simulink model "TWLan"  (R2025a)
settings: Solver=ode4  StartTime=0.0  StopTime=inf  FixedStep=0.01  RelTol=1e-3
libraries: AFCToolbox x9, simulink x3, etargetslib x2
settings Model: Creator=zqinghua  LastModifiedBy=zqhkd
settings OptimizationCC: DefaultParameterBehavior=Inlined  EnhancedBackFolding=on  PassReuseOutputArgsAs=Individual arguments  ZeroExternalMemoryAtStartup=off  ZeroInternalMemoryAtStartup=off  OptimizeBlockOrder=speed  DifferentSizesBufferReuse=on  OptimizationCustomize=off  EfficientTunableParamExpr=on
settings DebuggingCC: ParameterTunabilityLossMsg=error
settings HardwareCC: ProdBitPerInt=16.0  ProdBitPerPointer=16.0  ProdBitPerSizeT=16.0  ProdBitPerPtrDiffT=16.0  ProdLargestAtomicFloat=None  ProdWordSize=16.0  ProdHWDeviceType=STMicroelectronics->ST10/Super10
settings SFSimCC: MATLABDynamicMemAlloc=off
settings RTWCC: SystemTargetFile=AFCHawk.tlc  GenCodeOnly=on  TemplateMakefile=ert_default_tmf  GPUComputeCapability=3.5  Description=Embedded Coder
settings CodeAppCC: ForceParamTrailComments=on  IgnoreCustomStorageClasses=off  OperatorAnnotations=on  SimulinkDataObjDesc=on  SFDataObjDesc=on  InsertBlockDesc=on
settings STFCustomTargetCC: SystemTargetFile=AFCHawk.tlc  TargetLangStandard=C99 (ISO)  MultiwordLength=256.0  DynamicStringBufferSize=256.0  ModelReferenceCompliant=off  CombineOutputUpdateFcns=on  ERTCustomFileBanners=on  SupportContinuousTime=off  SupportNonInlinedSFcns=off  RemoveResetFunc=on  MATLABClassNameForMDSCustomization=Simulink.SoftwareTarget.ERTCustomization  GRTInterface=off  t_comPort=6.0  t_productKey=45638.0  t_comBaud=115200.0  t_BuildCPrj2Hex=on  t_productId=1.0  t_userCode=11120.0  t_DownLoad2Target=on
settings ERTTargetCC: ExtModeTransport=0.0  ExtModeStaticAlloc=off  ExtModeMexFile=ext_comm  ExtModeIntrfLevel=Level1  ERTCustomFileTemplate=example_file_process.tlc  DynamicArrayContainerType=coder::array  TargetLangStandard=C99 (ISO)  ModelReferenceCompliant=off  ParMdlRefBuildCompliant=off  CompOptLevelCompliant=off  ConcurrentExecutionCompliant=off  ModelStepFunctionPrototypeControlCompliant=off  CPPClassGenCompliant=off  UseToolchainInfoCompliant=off

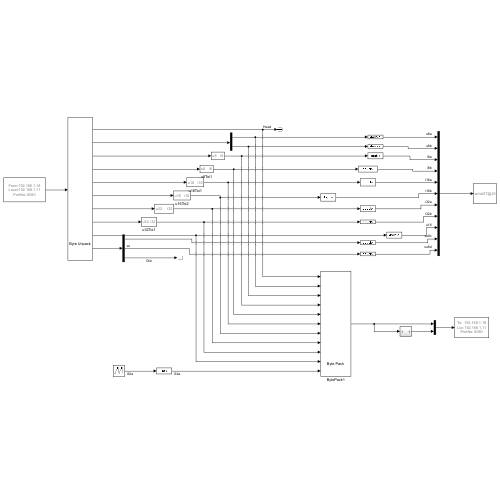
[thumbnail: Simulink's stored preview of the top-level diagram]
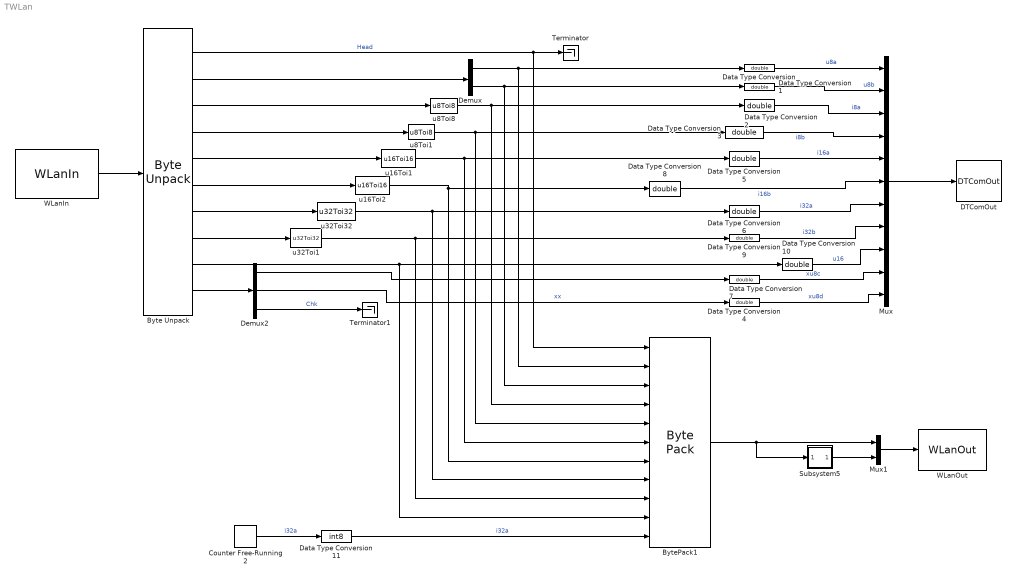
== system TWLan ==
  Byte Unpack : etargetslib/Byte Unpack  dimensions={1,2,1,1,1,1,1,1,1,3}  datatypes={'uint16','uint8','int8','int8','int16','int16','int32','int32','uint16','uint8'}  byteAlign=1
      settings: LibrarySourceBlock=embeddedtargetslib/Host Communication/Byte Unpack
  BytePack1 : etargetslib/Byte Pack  datatypes={'uint16','uint8','uint8','int8','int8','int16','int16','int32','int32','uint16','int8'}  byteAlign=1
  Counter Free-Running2 : simulink/Sources/Counter Free-Running  NumBits=8  tsamp=-1
  DTComOut : AFCToolbox/DeviceModule/DTComOut  Priority=8  g_frameType=20  g_outFreq=50  g_comPort=0  g_instName=0  g_id=0
      settings: SourceProductName=AFCToolbox
  Data Type Conversion{,1..10} (11 alike) : DataTypeConversion  OutDataTypeStr=double  SaturateOnIntegerOverflow=off  RndMeth=Floor
  Data Type Conversion11 : DataTypeConversion  OutDataTypeStr=int8  SaturateOnIntegerOverflow=off  RndMeth=Floor
  Demux : Demux  Outputs=2
  Demux2 : Demux  Outputs=3
  Mux : Mux  Inputs=11
  Mux1 : Mux  Inputs=2
  Subsystem5 : Subsystem
  Terminator : Terminator
  Terminator1 : Terminator
  WLanIn : AFCToolbox/DeviceModule/WLanIn  Priority=2  g_sampleTime=0.01  g_ipAddress=192.168.1.18  g_localIpAddress=192.168.1.11  g_iPort=8080  g_dataSize=23
      settings: SourceProductName=AFCToolbox
  WLanOut : AFCToolbox/DeviceModule/WLanOut  Priority=8  g_ipAddress=192.168.1.18  g_localIpAddress=192.168.1.11  g_iPort=8080  g_outFreq=1
      settings: SourceProductName=AFCToolbox
  u16Toi1 : AFCToolbox/APPModule/u16Toi16
      settings: SourceProductName=AFCToolbox
  u16Toi2 : AFCToolbox/APPModule/u16Toi16
      settings: SourceProductName=AFCToolbox
  u32Toi1 : AFCToolbox/APPModule/u32Toi32
      settings: SourceProductName=AFCToolbox
  u32Toi32 : AFCToolbox/APPModule/u32Toi32
      settings: SourceProductName=AFCToolbox
  u8Toi1 : AFCToolbox/APPModule/u8Toi8
      settings: SourceProductName=AFCToolbox
  u8Toi8 : AFCToolbox/APPModule/u8Toi8
      settings: SourceProductName=AFCToolbox
  wires:
  Byte Unpack/2 -> Demux/1
  Byte Unpack/3 -> u8Toi8/1
  Data Type Conversion8/1 -> Mux/6  "i16b"
  Demux2/1 -> Data Type Conversion7/1
  Data Type Conversion7/1 -> Mux/10  "xu8c"
  Demux2/2 -> Data Type Conversion4/1  "xx"
  Data Type Conversion2/1 -> Mux/3  "i8a"
  Data Type Conversion3/1 -> Mux/4  "i8b"
  Data Type Conversion6/1 -> Mux/7  "i32a"
  Demux/2 -> BytePack1/3, Data Type Conversion1/1
  Data Type Conversion/1 -> Mux/1  "u8a"
  Byte Unpack/4 -> u8Toi1/1
  Byte Unpack/1 -> BytePack1/1, Terminator/1  "Head"
  Demux/1 -> BytePack1/2, Data Type Conversion/1
  WLanIn/1 -> Byte Unpack/1
  Data Type Conversion1/1 -> Mux/2  "u8b"
  Mux/1 -> DTComOut/1
  Byte Unpack/10 -> Demux2/1
  Data Type Conversion5/1 -> Mux/5  "i16a"
  Byte Unpack/6 -> u16Toi2/1
  Byte Unpack/7 -> u32Toi32/1
  Byte Unpack/8 -> u32Toi1/1
  Byte Unpack/9 -> BytePack1/10, Data Type Conversion10/1
  Data Type Conversion9/1 -> Mux/8  "i32b"
  Data Type Conversion10/1 -> Mux/9  "u16"
  u8Toi8/1 -> BytePack1/4, Data Type Conversion2/1
  u8Toi1/1 -> BytePack1/5, Data Type Conversion3/1
  u16Toi1/1 -> BytePack1/6, Data Type Conversion5/1
  u32Toi32/1 -> BytePack1/8, Data Type Conversion6/1
  u32Toi1/1 -> BytePack1/9, Data Type Conversion9/1
  Data Type Conversion4/1 -> Mux/11  "xu8d"
  BytePack1/1 -> Subsystem5/1(In1), Mux1/1
  Subsystem5/1(Out1) -> Mux1/2
  Mux1/1 -> WLanOut/1
  Byte Unpack/5 -> u16Toi1/1
  u16Toi2/1 -> Data Type Conversion8/1, BytePack1/7
  Demux2/3 -> Terminator1/1  "Chk"
  Counter Free-Running2/1 -> Data Type Conversion11/1  "i32a"
  Data Type Conversion11/1 -> BytePack1/11  "i32a"

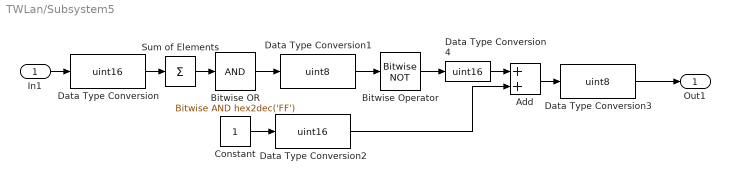
== system TWLan/Subsystem5 ==
  In1 : Inport
  Add : Sum
  Bitwise Operator : simulink/Logic and Bit Operations/Bitwise Operator  logicop=NOT  UseBitMask=off  BitMask=bin2dec('11011001')  BitMaskRealWorld=Stored Integer
  Bitwise OR : simulink/Logic and Bit Operations/Bitwise Operator  logicop=AND  UseBitMask=on  BitMask=hex2dec('FF')  BitMaskRealWorld=Stored Integer
  Constant : Constant
  Data Type Conversion : DataTypeConversion  OutDataTypeStr=uint16  SaturateOnIntegerOverflow=off  RndMeth=Floor
  Data Type Conversion1 : DataTypeConversion  OutDataTypeStr=uint8  SaturateOnIntegerOverflow=off  RndMeth=Floor
  Data Type Conversion2 : DataTypeConversion  OutDataTypeStr=uint16  SaturateOnIntegerOverflow=off  RndMeth=Floor
  Data Type Conversion3 : DataTypeConversion  OutDataTypeStr=uint8  SaturateOnIntegerOverflow=off  RndMeth=Floor
  Data Type Conversion4 : DataTypeConversion  OutDataTypeStr=uint16  SaturateOnIntegerOverflow=off  RndMeth=Floor
  Sum of Elements : Sum  Inputs=+
  Out1 : Outport
  wires:
  Data Type Conversion3/1 -> Out1/1
  Sum of Elements/1 -> Bitwise OR/1
  Bitwise OR/1 -> Data Type Conversion1/1
  Data Type Conversion/1 -> Sum of Elements/1
  Data Type Conversion1/1 -> Bitwise Operator/1
  In1/1 -> Data Type Conversion/1
  Bitwise Operator/1 -> Data Type Conversion4/1
  Constant/1 -> Data Type Conversion2/1
  Data Type Conversion2/1 -> Add/2
  Add/1 -> Data Type Conversion3/1
  Data Type Conversion4/1 -> Add/1
